simulink model "RTR2"  (R2026b)
settings: Solver=ode113  StopTime=1000  RelTol=1e-8
settings Model: Creator=user  LastModifiedBy=phuryn

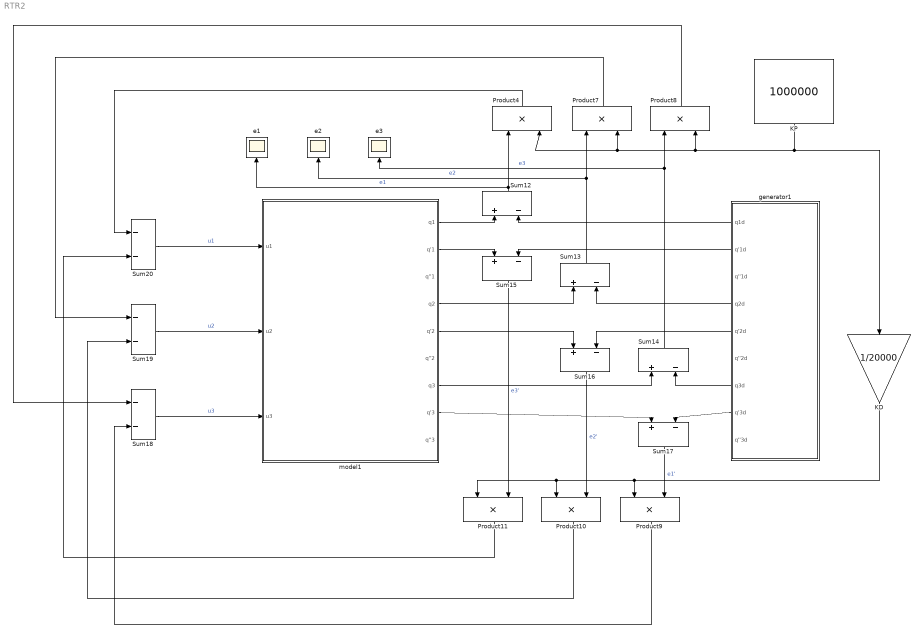
== system RTR2 ==
  KD : Gain  Gain=1/20000
  KP : Constant  Value=1000000
  Product{4,7..11} (6 alike) : Product
  Sum{12..17} (6 alike) : Sum  Inputs=+-
  Sum18 : Sum  Inputs=--
  Sum19 : Sum  Inputs=--
  Sum20 : Sum  Inputs=--
  e1 : Scope
      settings: ActiveDisplayYMinimum=-0.00017426146608073311  ActiveDisplayYMaximum=0.00017337443771042735  DataLoggingVariableName=ScopeData15
  e2 : Scope
      settings: ActiveDisplayYMinimum=-0.0010880394212289973  ActiveDisplayYMaximum=0.00021800949593887571  DataLoggingVariableName=ScopeData16
  e3 : Scope
      settings: ActiveDisplayYMinimum=-4.354511711385223E-5  ActiveDisplayYMaximum=-1.5104633608997737E-6  DataLoggingVariableName=ScopeData17
  generator1 : Subsystem
  model1 : Subsystem
  wires:
  model1/1(q1) -> Sum12/1
  generator1/1(q1d) -> Sum12/2
  model1/4(q2) -> Sum13/1
  generator1/4(q2d) -> Sum13/2
  generator1/7(q3d) -> Sum14/2
  model1/7(q3) -> Sum14/1
  model1/2(q'1) -> Sum15/1
  generator1/2(q'1d) -> Sum15/2
  model1/5(q'2) -> Sum16/1
  generator1/5(q'2d) -> Sum16/2
  generator1/8(q'3d) -> Sum17/2
  model1/8(q'3) -> Sum17/1
  Sum12/1 -> Product4/1, e1/1  "e1"
  Sum13/1 -> Product7/1, e2/1  "e2"
  Sum14/1 -> Product8/1, e3/1  "e3"
  Sum17/1 -> Product9/2  "e1'"
  Sum16/1 -> Product10/2  "e2'"
  Sum15/1 -> Product11/2  "e3'"
  KP/1 -> KD/1, Product4/2, Product7/2, Product8/2
  Sum18/1 -> model1/3(u3)  "u3"
  Sum19/1 -> model1/2(u2)  "u2"
  Sum20/1 -> model1/1(u1)  "u1"
  Product4/1 -> Sum20/1
  Product11/1 -> Sum20/2
  Product7/1 -> Sum19/1
  Product8/1 -> Sum18/1
  Product10/1 -> Sum19/2
  Product9/1 -> Sum18/2
  KD/1 -> Product9/1, Product10/1, Product11/1

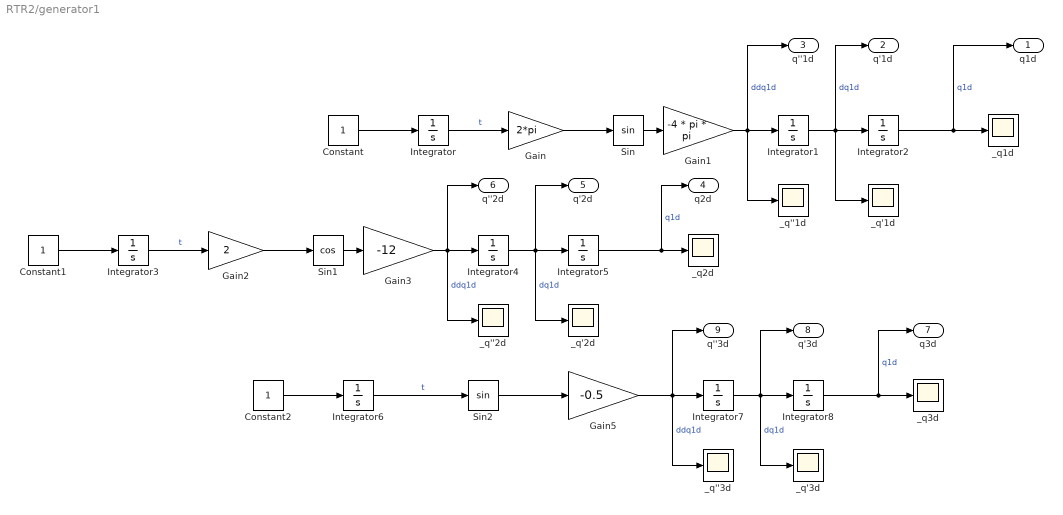
== system RTR2/generator1 ==
  Constant : Constant
  Constant1 : Constant
  Constant2 : Constant
  Gain : Gain  Gain=2*pi
  Gain1 : Gain  Gain=-4 * pi * pi
  Gain2 : Gain  Gain=2
  Gain3 : Gain  Gain=-12
  Gain5 : Gain  Gain=-0.5
  Integrator{,2..4,6,8} (6 alike) : Integrator
  Integrator1 : Integrator  InitialCondition=2 * pi
  Integrator5 : Integrator  InitialCondition=3
  Integrator7 : Integrator  InitialCondition=0.5
  Sin : Trigonometry
  Sin1 : Trigonometry  Operator=cos
  Sin2 : Trigonometry
  _q''1d : Scope
      settings: ActiveDisplayYMinimum=-1  ActiveDisplayYMaximum=1  DataLoggingVariableName=ScopeData8
  _q''2d : Scope
      settings: ActiveDisplayYMinimum=-48.709486010573571  ActiveDisplayYMaximum=48.709486010581045  DataLoggingVariableName=ScopeData9
  _q''3d : Scope
      settings: ActiveDisplayYMinimum=-48.709486010573571  ActiveDisplayYMaximum=48.709486010581045  DataLoggingVariableName=ScopeData12
  _q'1d : Scope
      settings: ActiveDisplayYMinimum=-6.3824112653345679  ActiveDisplayYMaximum=6.3464413266389137  DataLoggingVariableName=ScopeData7
  _q'2d : Scope
      settings: ActiveDisplayYMinimum=-6.3824112653345679  ActiveDisplayYMaximum=6.3464413266389137  DataLoggingVariableName=ScopeData10
  _q'3d : Scope
      settings: ActiveDisplayYMinimum=-6.3824112653345679  ActiveDisplayYMaximum=6.3464413266389137  DataLoggingVariableName=ScopeData13
  _q1d : Scope
      settings: ActiveDisplayYMinimum=0.9  ActiveDisplayYMaximum=1.1  DataLoggingVariableName=ScopeData6
  _q2d : Scope
      settings: ActiveDisplayYMinimum=2  ActiveDisplayYMaximum=4  DataLoggingVariableName=ScopeData11
  _q3d : Scope
      settings: ActiveDisplayYMinimum=-0.25541496120254592  ActiveDisplayYMaximum=2.2339894235166695  DataLoggingVariableName=ScopeData14
  q1d : Outport
  q'1d : Outport  Port=2
  q''1d : Outport  Port=3
  q2d : Outport  Port=4
  q'2d : Outport  Port=5
  "q''2d " : Outport  Port=6
  q3d : Outport  Port=7
  q'3d : Outport  Port=8
  q''3d : Outport  Port=9
  wires:
  Constant/1 -> Integrator/1
  Integrator/1 -> Gain/1  "t"
  Gain/1 -> Sin/1
  Sin/1 -> Gain1/1
  Gain1/1 -> q''1d/1, _q''1d/1, Integrator1/1  "ddq1d"
  Integrator1/1 -> q'1d/1, _q'1d/1, Integrator2/1  "dq1d"
  Integrator2/1 -> q1d/1, _q1d/1  "q1d"
  Gain2/1 -> Sin1/1
  Integrator5/1 -> q2d/1, _q2d/1  "q1d"
  Sin1/1 -> Gain3/1
  Constant1/1 -> Integrator3/1
  Integrator3/1 -> Gain2/1  "t"
  Integrator4/1 -> q'2d/1, _q'2d/1, Integrator5/1  "dq1d"
  Gain3/1 -> _q''2d/1, "q''2d "/1, Integrator4/1  "ddq1d"
  Integrator8/1 -> q3d/1, _q3d/1  "q1d"
  Sin2/1 -> Gain5/1
  Constant2/1 -> Integrator6/1
  Integrator6/1 -> Sin2/1  "t"
  Integrator7/1 -> q'3d/1, _q'3d/1, Integrator8/1  "dq1d"
  Gain5/1 -> q''3d/1, _q''3d/1, Integrator7/1  "ddq1d"

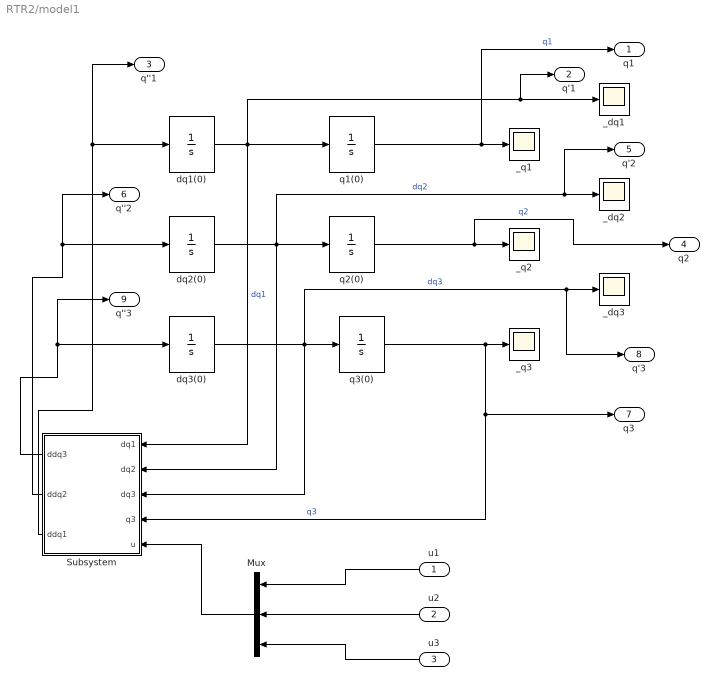
== system RTR2/model1 ==
  u1 : Inport
  u2 : Inport  Port=2
  u3 : Inport  Port=3
  Mux : Mux  Inputs=3
  Subsystem : Subsystem
  _dq1 : Scope
      settings: ActiveDisplayYMinimum=-1  ActiveDisplayYMaximum=1  DataLoggingVariableName=ScopeData3
  _dq2 : Scope
      settings: ActiveDisplayYMinimum=-1  ActiveDisplayYMaximum=1  DataLoggingVariableName=ScopeData4
  _dq3 : Scope
      settings: ActiveDisplayYMinimum=-1  ActiveDisplayYMaximum=1  DataLoggingVariableName=ScopeData5
  _q1 : Scope
      settings: ActiveDisplayYMinimum=-0.1597426040833444  ActiveDisplayYMaximum=-0.0015718859113596495
  _q2 : Scope
      settings: ActiveDisplayYMinimum=-0.0083845802473266479  ActiveDisplayYMaximum=-7.06681406811439E-5
  _q3 : Scope
      settings: ActiveDisplayYMinimum=-1  ActiveDisplayYMaximum=1  DataLoggingVariableName=ScopeData2
  dq1(0) : Integrator
  dq2(0) : Integrator
  dq3(0) : Integrator
  q1(0) : Integrator
  q2(0) : Integrator
  q3(0) : Integrator
  q1 : Outport
  q'1 : Outport  Port=2
  q''1 : Outport  Port=3
  q2 : Outport  Port=4
  q'2 : Outport  Port=5
  q''2 : Outport  Port=6
  q3 : Outport  Port=7
  q'3 : Outport  Port=8
  q''3 : Outport  Port=9
  wires:
  u3/1 -> Mux/3
  dq2(0)/1 -> Subsystem/2(dq2), q2(0)/1, q'2/1, _dq2/1  "dq2"
  Subsystem/1(ddq3) -> q''3/1, dq3(0)/1
  dq1(0)/1 -> Subsystem/1(dq1), q'1/1, _dq1/1, q1(0)/1  "dq1"
  q3(0)/1 -> q3/1, Subsystem/4(q3), _q3/1  "q3"
  q1(0)/1 -> q1/1, _q1/1  "q1"
  dq3(0)/1 -> Subsystem/3(dq3), q'3/1, _dq3/1, q3(0)/1  "dq3"
  Subsystem/2(ddq2) -> q''2/1, dq2(0)/1
  Subsystem/3(ddq1) -> q''1/1, dq1(0)/1
  q2(0)/1 -> q2/1, _q2/1  "q2"
  u1/1 -> Mux/1
  Mux/1 -> Subsystem/5(u)
  u2/1 -> Mux/2

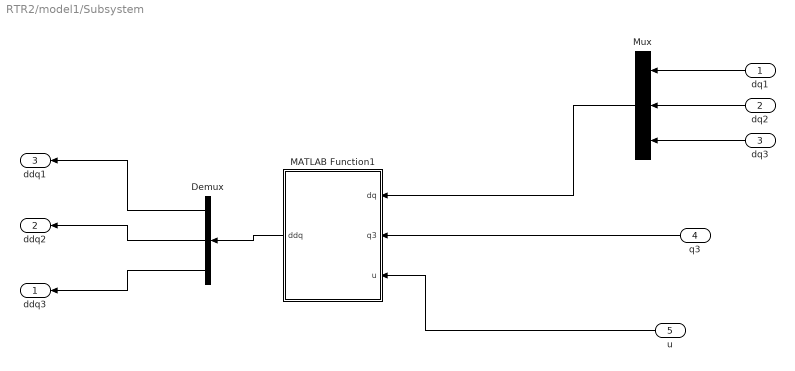
== system RTR2/model1/Subsystem ==
  dq1 : Inport
  dq2 : Inport  Port=2
  dq3 : Inport  Port=3
  q3 : Inport  Port=4
  u : Inport  Port=5
  Demux : Demux  Outputs=3
  MATLAB Function1 : MATLAB Function  TreatAsAtomicUnit=on
  Mux : Mux  Inputs=3
  ddq3 : Outport
  ddq2 : Outport  Port=2
  ddq1 : Outport  Port=3
  wires:
  dq1/1 -> Mux/1
  u/1 -> MATLAB Function1/3(u)
  q3/1 -> MATLAB Function1/2(q3)
  dq2/1 -> Mux/2
  dq3/1 -> Mux/3
  Mux/1 -> MATLAB Function1/1(dq)
  MATLAB Function1/1(ddq) -> Demux/1
  Demux/2 -> ddq2/1
  Demux/1 -> ddq1/1
  Demux/3 -> ddq3/1

== matlab function RTR2/model1/Subsystem/MATLAB Function1 ==
  data: ddq output size=3; dq input; q3 input; u input
function ddq = fcn(dq, q3, u)
dq1 = dq(1);
dq2 = dq(2);
dq3 = dq(3);
c3 = cos(q3);
s3 = sin(q3);

%======================================
% Macierz inercji
M11 = 2.4 + (0.8/3) * c3^2 + 1.2 * c3;
M22 = 40;
M23 = 0.6 * c3;
M33 = 0.8/3;
M = [M11,   0,   0;
    0, M22, M23;
    0, M23, M33];

%======================================
% Macierz Coriolisa
I = 0.6 * s3 + (0.8/3) * s3 * c3;
C11 = -dq3 * I;
C13 = -dq1 * I;
C23 = -dq3 * 0.6 * s3;
C31 =  dq1 * I;
C = [C11, 0, C13;
    0, 0, C23;
    C31, 0,   0];

%======================================
% Wektor grawitacji
D = [0; 392.4; 19.62 * c3];

%======================================
% Wektor przyspieszeń (3x1)
ddq = M \ (u - C * dq - D);
end
